simulink model "baseline_model"  (R2026b)
settings: Solver=ode3  StopTime=.035  FixedStep=Ts
model workspace (MAT data in the model file):
  Cf = 1.06653877518e-07
  Cout = 0.0022
  Cp = 2.2319584622e-08
  Cs = 1.84570546919e-08
  ESRf = 0.003
  ESRp = 0.005
  ESRs = 0.005
  Goff = 1e-08
  Ki = 15
  Kp = 0.012
  Lf = 3.8e-06
  Lmat = [2.19582561429e-05 -4.36667057516e-08 -2.64487562385e-10 -2.91825501354e-11 1.6585415982e-06 -4.36667057516e-08 2.19582561429e-05 -4.36667057516e-08 -2.64487562385e-10 1.6585415982e-06 -2.64487562385e-10 -4.36667057516e-08 ... (25 elements, 5x5)]
  RL = 3
  Rcoil = 0.019579897138
  Rf = 0.012
  RonSR = 0.0032
  RonTx = 0.01072
  Ts = 1e-08
  Vdc = 100
  Vtarget = 60
  bodyRon = 0.01
  bodyVf = 0.8
  deadTime = 4e-08
  f = 250000
  initialOutputVoltage = 0
  position = 0.9144
  softStart = 0.02
  srDeadTime = 4e-08
  srEnabled = 1
  srThreshold = 0.25
  u_nom = [0.70005165965 0.70005165965 0 0]
libraries: fl_lib x52, nesl_utility x42, ee_lib x20, ddtrack_lib x1
(part 4 of 4)

== system baseline_model/Section 4 bridge and LCC/Q4 ==
  g : Inport
  Data Type Conversion : DataTypeConversion  OutDataTypeStr=double  SaturateOnIntegerOverflow=off  RndMeth=Floor
  MOSFET : ee_lib/Semiconductors & Converters/MOSFET (Ideal, Switching)  port_option=ee.enum.controlport.ps  Rds=RonTx Ohm  Goff=Goff 1/Ohm  Vth=0.5 V  diode_param=2  diode_Vf=bodyVf V  diode_Ron=bodyRon Ohm  diode_Goff=Goff 1/Ohm  diode_C=5e-8 F  diode_iRM=-235 A  diode_iF=300 A  diode_idot=-50 A/us  diode_trr_param=1  diode_trr_factor=3  diode_trr=15 us  diode_Qrr=1.5e+3 s*uA  ids_specify=off  ids_priority=None  ids=0 A  ids_nominal_specify=off  ids_nominal_value=1  ids_nominal_unit=A  vds_specify=off  vds_priority=None  vds=0 V  vds_nominal_specify=off  vds_nominal_value=1  vds_nominal_unit=V  vgs_specify=off  vgs_priority=None  vgs=0 V  vgs_nominal_specify=off  vgs_nominal_value=1  vgs_nominal_unit=V  thermal_loss_option=ee.enum.converters.thermalLossOption.constantvalues  Von_data=[0, 1.1, 1.3, 1.45, 1.75, 2.25, 2.7; 0, 1, 1.15, 1.35, 1.7, 2.35, 3] V  Tj=[298.15, 398.15] K  Iout_data=[0, 10, 50, 100, 200, 400, 600] A  tabulateWithVds=false  Eon_data=[0, .29, 1.43, 2.86, 5.71, 13.14, 22.86; 0, .57, 2.63, 5.14, 10.29, 20.57, 30.29] * 1e-3 J  Eoff_data=[0, .21, 1.07, 2.14, 4.29, 9.86, 17.14; 0, .43, 1.97, 3.86, 7.71, 15.43, 22.71] * 1e-3 J  Eon_data_3D=[zeros(2, 5, 3)] J  Eoff_data_3D=[zeros(2, 5, 3)] J  Tj_loss=[298.15, 448.15] K  Iout_data_loss=[0, 10, 20, 30, 40] A  Vds_loss=[0, 150, 300] V  Eon_scalar=22.86e-3 J  Eoff_scalar=17.14e-3 J  Voff=300 V  Iout_scalar=600 A  useCurrentFromPreviousCycle=true  currentMeasDelay=0 s  useVoltageFromPreviousCycle=true  voltageMeasDelay=0 s  diodeModelType=ee.enum.converters.diodeModelType.pwl  diodeTableType=ee.enum.diode.tableType.IfMat  diode_ReverseIVType=ee.enum.diode.diodeReverseIV.constant  diode_IfMat=[.07, .12, .19, 1.75, 4.24, 7.32, 11.2; .16, .3, .72, 2.14, 4.02, 6.35, 9.12] A  diode_VfMat=[.9, 1.15, 1.25, 1.5, 1.75, 2.17, 2.6, 2.85; .58, .68, .75, 1.1, 1.38, 1.77, 2.27, 2.7] V  diode_TjVec=[25, 125] degC  diode_VfVec=[.5, .7, .9, 1.3, 1.7, 2.1, 2.5] V  diode_IfVec=[.1, .2, .5, 1, 2, 4, 7, 10] A  diode_IrMat=[1e-06, 2e-06, 5e-06, 1e-05, 2.5e-05, 5e-05, .0001; 2e-06, 5e-06, 1e-05, 4e-05, 8e-05, .0002, .0005] A  diode_VrMat=[10, 100, 200, 250, 300, 325, 350; 10, 70, 160, 220, 270, 300, 320] V  diode_VrVec=[10, 20, 40, 50, 70, 80, 100] V  diode_IrVec=[1e-06, 2e-06, 5e-06, 1e-05, 2e-05, 5e-05, .0001] A  diode_Vr=-600 V  diode_Ls=150 nH  diode_Erec=0.03 J  diode_rec_loss_model=ee.enum.diode.reverseRecoveryModelTabulateUpTo3D.fixed  diode_ErecVal=0 J  diode_scaleWithIandV=true  diode_ErecMat=zeros(2, 3) J  diodeErecMat3D=zeros(2, 3, 2) J  diode_TjrecVec=[298.15, 398.15] K  diode_IfrecVec=[.1, 1, 10] A  diodeVrecVec=[0, 100] V  diode_IrecVal=10 A  diode_VrecVal=10 V  diode_tFilter=1 / 1000 / 100 s  separateThermalPortForDiode=false  thermal_network_parameterization=ee.enum.thermalNetworkTopology.external  Rth=[.03, .2] K/W  Rth_Cauer=[.03, .1, .2] K/W  Rth_Foster=[.03, .2] K/W  thermal_mass_parameterization=ee.enum.thermalNetwork.timeconstant  thermal_mass=[3, 25] J/K  thermal_mass_Cauer=[3, 10, 25] J/K  thermal_mass_Foster=[33, 50] J/K  thermal_time_constant=[.1, 5] s  thermal_time_constant_Cauer=[.1, 1, 5] s  thermal_time_constant_Foster=[1, 10] s  thermal_mass_initial_temperatures=[25, 25] degC  thermal_mass_initial_temperatures_Cauer=[25, 25, 25] degC  junction_thermal_mass=0.1 J/K  Tvec_initial_Foster=[25, 25, 25, 25] degC  RthDiode=[.03, .2] K/W  RthCauerDiode=[.03, .1, .2] K/W  RthFosterDiode=[.03, .2] K/W  thermalMassDiode=[3, 25] J/K  thermalMassCauerDiode=[3, 10, 25] J/K  thermalMassFosterDiode=[33, 50] J/K  thermalTauDiode=[.1, 5] s  thermalTauCauerDiode=[.1, 1, 5] s  thermalTauFosterDiode=[1, 10] s  thermalMassInitTempDiode=[25, 25] degC  thermalMassInitTempCauerDiode=[25, 25, 25] degC  junctionthermalMassDiode=0.1 J/K  TVecInitialFosterDiode=[25, 25] degC  no_thermal_network=ee.enum.enable.no  mosfet_junction_temperature_specify=off  mosfet_junction_temperature_priority=None  mosfet_junction_temperature=25 degC  mosfet_junction_temperature_nominal_specify=off  mosfet_junction_temperature_nominal_value=1  mosfet_junction_temperature_nominal_unit=degC  diode_junction_temperature_specify=off  diode_junction_temperature_priority=None  diode_junction_temperature=25 degC  diode_junction_temperature_nominal_specify=off  diode_junction_temperature_nominal_value=1  diode_junction_temperature_nominal_unit=degC  Qj_specify=off  Qj_priority=None  Qj=0 W  Qj_nominal_specify=off  Qj_nominal_value=1  Qj_nominal_unit=W  accumulatedSwitchingLosses_specify=off  accumulatedSwitchingLosses_priority=None  accumulatedSwitchingLosses=0 J
  Simulink-PS Converter : nesl_utility/Simulink-PS Converter  PhysicalDomain=network_engine_domain  SubClassName=ps_input  LeftPortType=input  RightPortType=output  PseudoPeriodic=off  Frequencies=[]  NoiseDistribution=none  NoiseParameters=[]  Unit=1  AffineConversion=off  FilteringAndDerivatives=provide  SimscapeFilterOrder=1  InputFilterTimeConstant=0.001  UdotUserProvided=0
  D : PMIOPort  Side=Left
  S : PMIOPort  Port=2  Side=Right
  wires:
  Data Type Conversion/1 -> Simulink-PS Converter/1
  g/1 -> Data Type Conversion/1
  connections:
  MOSFET/RConn1 -- D/RConn1
  Simulink-PS Converter/RConn1 -- MOSFET/LConn1
  S/RConn1 -- MOSFET/RConn2

== matlab function baseline_model/SR controller ==
  data: current input; positive output; negative output; Ts parameter; srDeadTime parameter; srThreshold parameter; srEnabled parameter
function [positive,negative] = sr_control(current, Ts, srDeadTime, srThreshold, srEnabled)
%#codegen
% Parameters: Ts, srDeadTime, srThreshold, srEnabled.
% Input is delayed one sample to avoid a physical-network algebraic loop.
% Turn off near zero current; require a stable polarity before turning on.
persistent previous stable
if isempty(previous)
    previous=0; stable=0;
end
polarity=0;
if current>srThreshold
    polarity=1;
elseif current<-srThreshold
    polarity=-1;
end
if polarity~=previous || polarity==0
    stable=0;
else
    stable=min(stable+1,ceil(srDeadTime/Ts)+1);
end
previous=polarity;
ready=stable>=ceil(srDeadTime/Ts) && srEnabled>0;
positive=double(ready && polarity==1);
negative=double(ready && polarity==-1);
end

== matlab function baseline_model/Four bridge controller ==
  data: t input; g output; v input; modulation output; reference output; f parameter; Ts parameter; Vtarget parameter; softStart parameter; deadTime parameter; Kp parameter; Ki parameter; u_nom parameter
function [g, modulation, reference] = pwm_track(t,v, f, Ts, Vtarget, softStart, deadTime, Kp, Ki, u_nom)
%#codegen
% Common fundamental phase across all four phase-shifted full bridges.
% Each bridge's complementary pair has enforced break-before-make.
persistent integral lastcycle command previous offcount
if isempty(integral)
 integral=0;lastcycle=-1;command=0;previous=zeros(16,1);offcount=ones(16,1)*1e6;
end
N=round(1/(f*Ts));tick=round(t/Ts);cycle=floor(tick/N);phase=mod(tick,N);
reference=Vtarget*min(t/softStart,1);
if cycle~=lastcycle
 error=reference-v;raw=reference/Vtarget+Kp*error+integral;
 if (raw<1/max(u_nom) && raw>0) || (raw>=1/max(u_nom) && error<0) || (raw<=0 && error>0)
  integral=integral+Ki*error/f;
 end
 command=max(0,min(1/max(u_nom),reference/Vtarget+Kp*error+integral));lastcycle=cycle;
end
modulation=min(1,max(0,u_nom(:)*command));desired=zeros(16,1);
dead=ceil(deadTime/Ts);
for k=1:4
 idx=4*(k-1);m=modulation(k);
 if m<.003
  desired(idx+2)=1;desired(idx+4)=1; % zero-vector clamp; tanks remain connected
 else
  halfwidth=round(N*asin(m)/(2*pi));
  a=mod(phase-(N/4-halfwidth),N);b=mod(phase-(N/4+halfwidth),N);
  desired(idx+1)=double(a>=dead && a<N/2);desired(idx+2)=double(a>=N/2+dead);
  desired(idx+3)=double(b>=dead && b<N/2);desired(idx+4)=double(b>=N/2+dead);
 end
end
g=zeros(16,1);
for j=1:16
 partner=j+1;if mod(j,2)==0,partner=j-1;end
 if previous(j)==0,offcount(j)=min(offcount(j)+1,1e6);else,offcount(j)=0;end
 if desired(j)>0 && desired(partner)==0 && previous(partner)==0 && offcount(partner)>=dead
  g(j)=1;
 end
end
previous=g;
end
